simulink model "ARDroneHover_V2_ALTER_D"  (R2026a)
settings: Solver=ode1  StopTime=Inf  FixedStep=sampleTime  EnableMultiTasking=on
values from neighbouring files (symbols this model uses):
  sampleTime = 1/200    (= 0.005)    [Copy_of_setupHover_EXEC_D.m]    (also in Copy_of_setupHover_EXEC_E.m; setupHover.m; setupWPTracking.m)
undefined symbols (not defined in the file or in its folder): Standard_Devices, UDP_Protocol
libraries: sldrtlib x3, dspnetwork x3, aerolibanimutils x1
settings Model: ExtModeTrigDuration=100000  Creator=Paul  LastModifiedBy=vicqu
settings DataIOCC: SignalLoggingSaveFormat=ModelDataLogs  TimeSaveName=time
settings OptimizationCC: InitFltsAndDblsToZero=on
settings DebuggingCC: UnderspecifiedInitializationDetection=Classic
settings HardwareCC: ProdBitPerLong=64.0  ProdHWDeviceType=Intel->x86-64 (Mac OS X)
settings RTWCC: SystemTargetFile=sldrt.tlc  TemplateMakefile=sldrt.tmf  RTWCompilerOptimization=on  Description=Simulink Desktop Real-Time
settings CodeAppCC: MaxIdLength=95.0
settings STFCustomTargetCC: SystemTargetFile=sldrt.tlc  MultiwordLength=2048.0  ModelReferenceCompliant=off  MATLABClassNameForMDSCustomization=Simulink.SoftwareTarget.TargetSpecificTriggerConfigurationBase
settings SimulinkDesktopRealTimeCC: TargetPreCompLibLocation=/Applications/MATLAB_R2017b.app/toolbox/sldrt/lib/maci64  TargetLangStandard=C89/C90 (ANSI)  SupportVariableSizeSignals=off

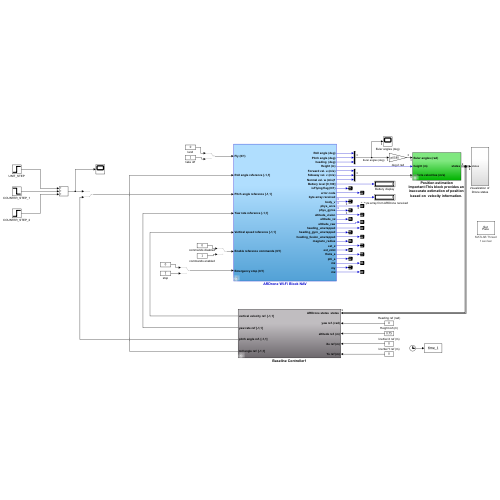
[thumbnail: Simulink's stored preview of the top-level diagram]
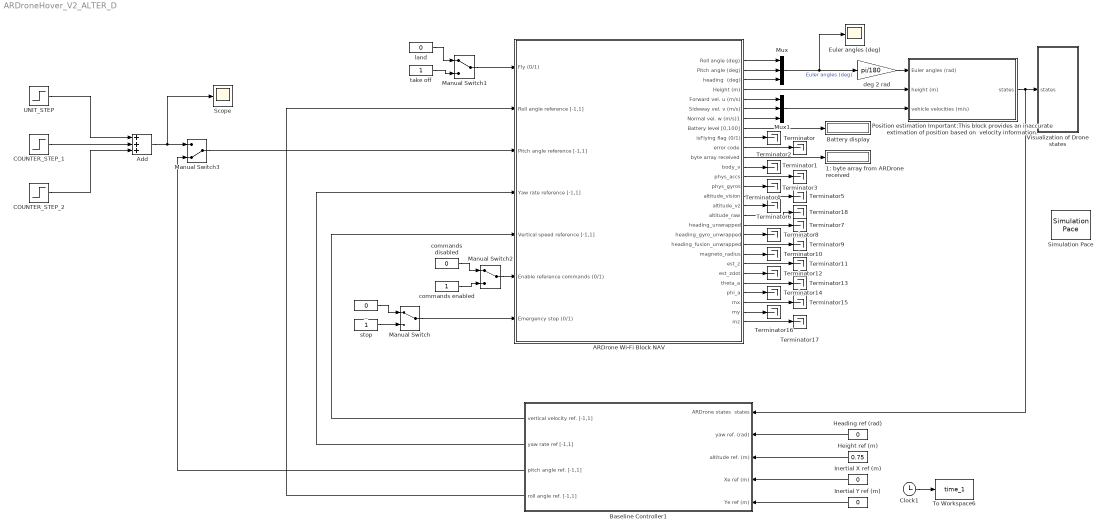
== system ARDroneHover_V2_ALTER_D ==
  "1: byte array from ARDrone received " : Display
  ARDrone Wi-Fi Block NAV : Subsystem  AncestorBlock=ARBlocks/ARDrone Wi-Fi Block NAV
  Add : Sum  Inputs=+++
  Baseline Controller1 : Subsystem  AncestorBlock=ARBlocks/Baseline Controller
  Battery display : Display
  COUNTER_STEP_1 : Step  Time=24  FinalValue=-2  SampleTime=0
  COUNTER_STEP_2 : Step  Time=28  SampleTime=0
  Clock1 : Clock
  Euler angles (deg) : Scope
      settings: ActiveDisplayYMinimum=-141.77037  ActiveDisplayYMaximum=21.99337  DataLoggingMaxPoints=500000
  Heading ref (rad) : Constant  Value=0
  Height ref (m) : Constant  Value=0.75
  Inertial X ref (m) : Constant  Value=0
  Inertial Y ref (m) : Constant  Value=0
  Manual Switch : ManualSwitch
  Manual Switch1 : ManualSwitch
  Manual Switch2 : ManualSwitch
  Manual Switch3 : ManualSwitch  CurrentSetting=0
  Mux : Mux  Inputs=3
  Mux1 : Mux  Inputs=3
  "Position estimation Important:This block provides an inaccurate extimation of position based on  velocity information. " : Subsystem  AncestorBlock=|
      | ARBlocks/Position estimation
      | Important:This block provides an 
      | inaccurate extimation of position 
      | based on  velocity information.
  Scope : Scope
      settings: ActiveDisplayYMinimum=-1  ActiveDisplayYMaximum=1
  Simulation Pace : aerolibanimutils/Simulation Pace  SimulationPace=1  SleepMode=MATLAB Thread  OutputPaceError=off  SampleTime=sampleTime
  Terminator{,1..18} (19 alike) : Terminator
  To Workspace6 : ToWorkspace  VariableName=time_1  SampleTime=sampleTime
  UNIT_STEP : Step  Time=20  SampleTime=0
  Visualization of Drone states : Subsystem
  _ : Constant  Value=0
  commands disabled : Constant  Value=0
  commands enabled : Constant
  deg 2 rad : Gain  Gain=pi/180
  land : Constant  Value=0
  stop : Constant
  take off : Constant
  wires:
  _/1 -> Manual Switch/1
  stop/1 -> Manual Switch/2
  land/1 -> Manual Switch1/1
  take off/1 -> Manual Switch1/2
  commands disabled/1 -> Manual Switch2/1
  commands enabled/1 -> Manual Switch2/2
  Manual Switch1/1 -> ARDrone Wi-Fi Block NAV/1(Fly (0/1))
  Manual Switch2/1 -> ARDrone Wi-Fi Block NAV/6(Enable reference commands (0/1))
  Manual Switch/1 -> ARDrone Wi-Fi Block NAV/7(Emergency stop (0/1))
  ARDrone Wi-Fi Block NAV/1(Roll angle (deg)) -> Mux/1
  ARDrone Wi-Fi Block NAV/2(Pitch angle (deg)) -> Mux/2
  ARDrone Wi-Fi Block NAV/5(Forward vel. u (m/s)) -> Mux1/1
  ARDrone Wi-Fi Block NAV/6(Sideway vel. v (m/s)) -> Mux1/2
  ARDrone Wi-Fi Block NAV/7(Normal vel. w (m/s)1) -> Mux1/3
  Mux/1 -> deg 2 rad/1, Euler angles (deg)/1  "Euler angles (deg)"
  ARDrone Wi-Fi Block NAV/8(Battery level [0,100]) -> Battery display/1
  Baseline Controller1/1(vertical velocity ref. [-1,1]) -> ARDrone Wi-Fi Block NAV/5(Vertical speed reference [-1,1])
  "Position estimation Important:This block provides an inaccurate extimation of position based on  velocity information. "/1(states) -> Baseline Controller1/1("ARDrone states  states "), Visualization of Drone states/1(states)
  deg 2 rad/1 -> "Position estimation Important:This block provides an inaccurate extimation of position based on  velocity information. "/1(Euler angles (rad))
  ARDrone Wi-Fi Block NAV/4(Height (m)) -> "Position estimation Important:This block provides an inaccurate extimation of position based on  velocity information. "/2(height (m))
  Mux1/1 -> "Position estimation Important:This block provides an inaccurate extimation of position based on  velocity information. "/3(vehicle velocities (m/s))
  Baseline Controller1/4(roll angle ref. [-1,1]) -> ARDrone Wi-Fi Block NAV/2(Roll angle reference [-1,1])
  ARDrone Wi-Fi Block NAV/3(heading  (deg)) -> Mux/3
  ARDrone Wi-Fi Block NAV/9(isFlying flag (0/1)) -> Terminator/1
  ARDrone Wi-Fi Block NAV/10(error code) -> Terminator1/1
  ARDrone Wi-Fi Block NAV/11(byte array received) -> "1: byte array from ARDrone received "/1
  Baseline Controller1/2(yaw rate ref [-1,1]) -> ARDrone Wi-Fi Block NAV/4(Yaw rate reference [-1,1])
  Clock1/1 -> To Workspace6/1
  Height ref (m)/1 -> Baseline Controller1/3(altitude ref. (m))
  Inertial X ref (m)/1 -> Baseline Controller1/4(Xe ref (m))
  Inertial Y ref (m)/1 -> Baseline Controller1/5(Ye ref (m))
  Heading ref (rad)/1 -> Baseline Controller1/2(yaw ref. (rad))
  ARDrone Wi-Fi Block NAV/17(altitude_raw) -> Terminator18/1
  ARDrone Wi-Fi Block NAV/12(body_v) -> Terminator2/1
  ARDrone Wi-Fi Block NAV/13(phys_accs) -> Terminator3/1
  ARDrone Wi-Fi Block NAV/14(phys_gyros) -> Terminator4/1
  ARDrone Wi-Fi Block NAV/15(altitude_vision) -> Terminator5/1
  ARDrone Wi-Fi Block NAV/16(altitude_vz) -> Terminator6/1
  ARDrone Wi-Fi Block NAV/19(heading_gyro_unwrapped) -> Terminator8/1
  ARDrone Wi-Fi Block NAV/18(heading_unwrapped) -> Terminator7/1
  ARDrone Wi-Fi Block NAV/21(magneto_radius) -> Terminator10/1
  ARDrone Wi-Fi Block NAV/20(heading_fusion_unwrapped) -> Terminator9/1
  ARDrone Wi-Fi Block NAV/23(est_zdot) -> Terminator12/1
  ARDrone Wi-Fi Block NAV/22(est_z) -> Terminator11/1
  ARDrone Wi-Fi Block NAV/25(phi_a) -> Terminator14/1
  ARDrone Wi-Fi Block NAV/24(theta_a) -> Terminator13/1
  ARDrone Wi-Fi Block NAV/27(my) -> Terminator16/1
  ARDrone Wi-Fi Block NAV/26(mx) -> Terminator15/1
  ARDrone Wi-Fi Block NAV/28(mz) -> Terminator17/1
  Manual Switch3/1 -> ARDrone Wi-Fi Block NAV/3(Pitch angle reference [-1,1])
  Baseline Controller1/3(pitch angle ref. [-1,1]) -> Manual Switch3/2
  Add/1 -> Scope/1, Manual Switch3/1
  UNIT_STEP/1 -> Add/1
  COUNTER_STEP_1/1 -> Add/2
  COUNTER_STEP_2/1 -> Add/3

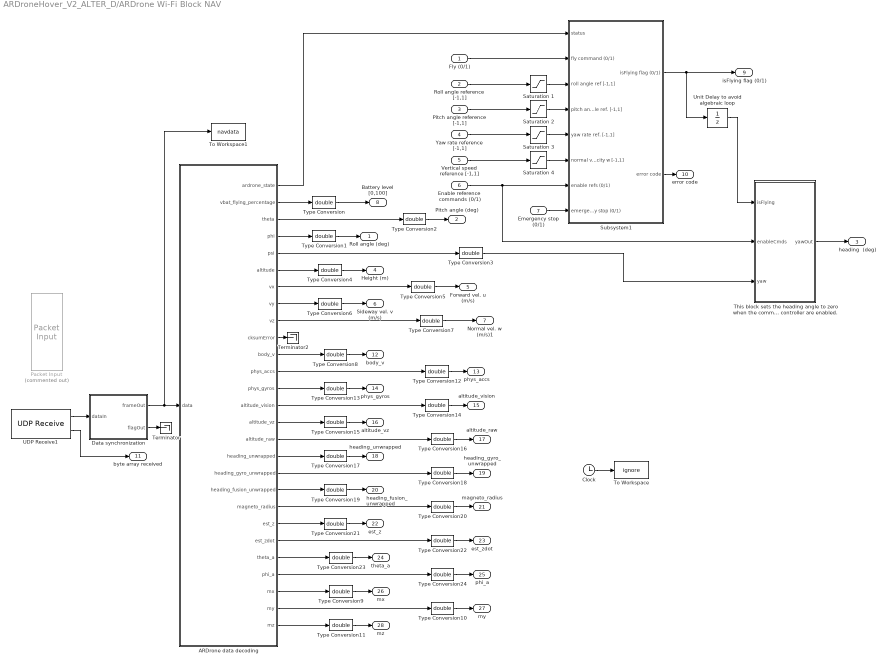
== system ARDroneHover_V2_ALTER_D/ARDrone Wi-Fi Block NAV ==
  Fly (0/1) : Inport
  Roll angle reference [-1,1] : Inport  Port=2
  Pitch angle reference [-1,1] : Inport  Port=3
  Yaw rate reference [-1,1] : Inport  Port=4
  Vertical speed reference [-1,1] : Inport  Port=5
  Enable reference commands (0/1) : Inport  Port=6
  Emergency stop (0/1) : Inport  Port=7
  ARDrone data decoding : MATLAB Function  TreatAsAtomicUnit=on
  Clock : Clock
      settings: Decimation=100
  "Data synchronization " : MATLAB Function  TreatAsAtomicUnit=on
  Packet Input : sldrtlib/Packet Input  Commented=on  SampleTime=sampleTime  MaxMissedTicks=100  ShowMissedTicks=off  YieldWhenWaiting=off  DrvName=Standard_Devices/UDP_Protocol  DrvAddress=5554  DrvOptions=[3232235777 5554]  PacketSize=2190  DataTypes='2190*uint8'  ShowReady=on  ShowError=off  PacketID=1  ByteOrder=1  ShowTimestamp=off
      settings: AttributesFormatString=UDP Protocol [5554]
  Saturation {1..4} (4 alike) : Saturate  UpperLimit=1  LowerLimit=-1
  Subsystem1 : Subsystem
  Terminator : Terminator
  Terminator2 : Terminator
  "This block sets the heading angle to zero when the commands from the Simulink controller are enabled. " : MATLAB Function  TreatAsAtomicUnit=on
  To Workspace : ToWorkspace  VariableName=ignore  SaveFormat=Timeseries  SampleTime=-1
  To Workspace1 : ToWorkspace  VariableName=navdata  SaveFormat=Structure With Time  SampleTime=-1
  Type Conversion{,1..24} (25 alike) : DataTypeConversion  OutDataTypeStr=double  SaturateOnIntegerOverflow=off  RndMeth=Floor
  UDP Receive1 : dspnetwork/UDP Receive  localURL='0.0.0.0'  localPort=5554  remoteURL='192.168.1.1'  remotePort=-1  recvBufferSize=8192  dims=2190  signalDatatype=uint8  isComplex=off  isVarSize=off  showBlockingTime=off  blockingTime=0  sampletime=sampleTime  blockPlatform=[]
  Unit Delay to avoid algebraic loop : UnitDelay  SampleTime=-1
  Roll angle (deg) : Outport  VectorParamsAs1DForOutWhenUnconnected=off
  Pitch angle (deg) : Outport  Port=2  VectorParamsAs1DForOutWhenUnconnected=off
  heading  (deg) : Outport  Port=3  VectorParamsAs1DForOutWhenUnconnected=off
  Height (m) : Outport  Port=4  VectorParamsAs1DForOutWhenUnconnected=off
  Forward vel. u (m/s) : Outport  Port=5  VectorParamsAs1DForOutWhenUnconnected=off
  Sideway vel. v (m/s) : Outport  Port=6  VectorParamsAs1DForOutWhenUnconnected=off
  Normal vel. w (m/s)1 : Outport  Port=7  VectorParamsAs1DForOutWhenUnconnected=off
  Battery level [0,100] : Outport  Port=8  VectorParamsAs1DForOutWhenUnconnected=off
  isFlying flag (0/1) : Outport  Port=9  VectorParamsAs1DForOutWhenUnconnected=off
  error code : Outport  Port=10  VectorParamsAs1DForOutWhenUnconnected=off
  byte array received : Outport  Port=11  VectorParamsAs1DForOutWhenUnconnected=off
  body_v : Outport  Port=12  VectorParamsAs1DForOutWhenUnconnected=off
  phys_accs : Outport  Port=13  VectorParamsAs1DForOutWhenUnconnected=off
  phys_gyros : Outport  Port=14  VectorParamsAs1DForOutWhenUnconnected=off
  altitude_vision : Outport  Port=15  VectorParamsAs1DForOutWhenUnconnected=off
  altitude_vz : Outport  Port=16  VectorParamsAs1DForOutWhenUnconnected=off
  altitude_raw : Outport  Port=17  VectorParamsAs1DForOutWhenUnconnected=off
  heading_unwrapped : Outport  Port=18  VectorParamsAs1DForOutWhenUnconnected=off
  heading_gyro_unwrapped : Outport  Port=19  VectorParamsAs1DForOutWhenUnconnected=off
  heading_fusion_unwrapped : Outport  Port=20  VectorParamsAs1DForOutWhenUnconnected=off
  magneto_radius : Outport  Port=21  VectorParamsAs1DForOutWhenUnconnected=off
  est_z : Outport  Port=22  VectorParamsAs1DForOutWhenUnconnected=off
  est_zdot : Outport  Port=23  VectorParamsAs1DForOutWhenUnconnected=off
  theta_a : Outport  Port=24  VectorParamsAs1DForOutWhenUnconnected=off
  phi_a : Outport  Port=25  VectorParamsAs1DForOutWhenUnconnected=off
  mx : Outport  Port=26  VectorParamsAs1DForOutWhenUnconnected=off
  my : Outport  Port=27  VectorParamsAs1DForOutWhenUnconnected=off
  mz : Outport  Port=28  VectorParamsAs1DForOutWhenUnconnected=off
  wires:
  ARDrone data decoding/27(mz) -> Type Conversion11/1
  Type Conversion11/1 -> mz/1
  ARDrone data decoding/26(my) -> Type Conversion10/1
  Type Conversion10/1 -> my/1
  ARDrone data decoding/25(mx) -> Type Conversion9/1
  Type Conversion9/1 -> mx/1
  ARDrone data decoding/24(phi_a) -> Type Conversion24/1
  ARDrone data decoding/23(theta_a) -> Type Conversion23/1
  ARDrone data decoding/22(est_zdot) -> Type Conversion22/1
  ARDrone data decoding/21(est_z) -> Type Conversion21/1
  ARDrone data decoding/20(magneto_radius) -> Type Conversion20/1
  ARDrone data decoding/19(heading_fusion_unwrapped) -> Type Conversion19/1
  ARDrone data decoding/18(heading_gyro_unwrapped) -> Type Conversion18/1
  ARDrone data decoding/17(heading_unwrapped) -> Type Conversion17/1
  ARDrone data decoding/16(altitude_raw) -> Type Conversion16/1
  ARDrone data decoding/15(altitude_vz) -> Type Conversion15/1
  ARDrone data decoding/14(altitude_vision) -> Type Conversion14/1
  ARDrone data decoding/13(phys_gyros) -> Type Conversion13/1
  ARDrone data decoding/12(phys_accs) -> Type Conversion12/1
  ARDrone data decoding/11(body_v) -> Type Conversion8/1
  ARDrone data decoding/10(cksumError) -> Terminator2/1
  ARDrone data decoding/9(vz) -> Type Conversion7/1
  ARDrone data decoding/8(vy) -> Type Conversion6/1
  ARDrone data decoding/7(vx) -> Type Conversion5/1
  ARDrone data decoding/6(altitude) -> Type Conversion4/1
  ARDrone data decoding/5(psi) -> Type Conversion3/1
  ARDrone data decoding/4(phi) -> Type Conversion1/1
  ARDrone data decoding/3(theta) -> Type Conversion2/1
  ARDrone data decoding/2(vbat_flying_percentage) -> Type Conversion/1
  Type Conversion24/1 -> phi_a/1
  Type Conversion23/1 -> theta_a/1
  Type Conversion22/1 -> est_zdot/1
  Type Conversion21/1 -> est_z/1
  Type Conversion20/1 -> magneto_radius/1
  Type Conversion19/1 -> heading_fusion_unwrapped/1
  Type Conversion18/1 -> heading_gyro_unwrapped/1
  Type Conversion17/1 -> heading_unwrapped/1
  Type Conversion16/1 -> altitude_raw/1
  Type Conversion15/1 -> altitude_vz/1
  Type Conversion14/1 -> altitude_vision/1
  Type Conversion13/1 -> phys_gyros/1
  Type Conversion12/1 -> phys_accs/1
  Type Conversion8/1 -> body_v/1
  Clock/1 -> To Workspace/1
  Unit Delay to avoid algebraic loop/1 -> "This block sets the heading angle to zero when the commands from the Simulink controller are enabled. "/1(isFlying)
  "Data synchronization "/2(flagOut) -> Terminator/1
  Saturation 4/1 -> Subsystem1/6(normal velocity w [-1,1])
  Saturation 3/1 -> Subsystem1/5(yaw rate ref. [-1,1])
  Saturation 2/1 -> Subsystem1/4(pitch angle ref. [-1,1])
  Saturation 1/1 -> Subsystem1/3(roll angle ref [-1,1])
  Fly (0/1)/1 -> Subsystem1/2(fly command (0/1))
  "This block sets the heading angle to zero when the commands from the Simulink controller are enabled. "/1(yawOut) -> heading  (deg)/1
  Type Conversion3/1 -> "This block sets the heading angle to zero when the commands from the Simulink controller are enabled. "/3(yaw)
  Type Conversion7/1 -> Normal vel. w (m/s)1/1
  Type Conversion6/1 -> Sideway vel. v (m/s)/1
  Type Conversion5/1 -> Forward vel. u (m/s)/1
  Type Conversion4/1 -> Height (m)/1
  Type Conversion2/1 -> Pitch angle (deg)/1
  Type Conversion1/1 -> Roll angle (deg)/1
  Type Conversion/1 -> Battery level [0,100]/1
  Subsystem1/2(error code) -> error code/1
  Subsystem1/1(isFlying flag (0/1)) -> Unit Delay to avoid algebraic loop/1, isFlying flag (0/1)/1
  Emergency stop (0/1)/1 -> Subsystem1/8(emergency stop (0/1))
  Enable reference commands (0/1)/1 -> Subsystem1/7(enable refs (0/1)), "This block sets the heading angle to zero when the commands from the Simulink controller are enabled. "/2(enableCmds)
  Vertical speed reference [-1,1]/1 -> Saturation 4/1
  Yaw rate reference [-1,1]/1 -> Saturation 3/1
  Pitch angle reference [-1,1]/1 -> Saturation 2/1
  Roll angle reference [-1,1]/1 -> Saturation 1/1
  ARDrone data decoding/1(ardrone_state) -> Subsystem1/1(status)
  UDP Receive1/2 -> byte array received/1
  "Data synchronization "/1(frameOut) -> To Workspace1/1, ARDrone data decoding/1(data)
  UDP Receive1/1 -> "Data synchronization "/1(dataIn)

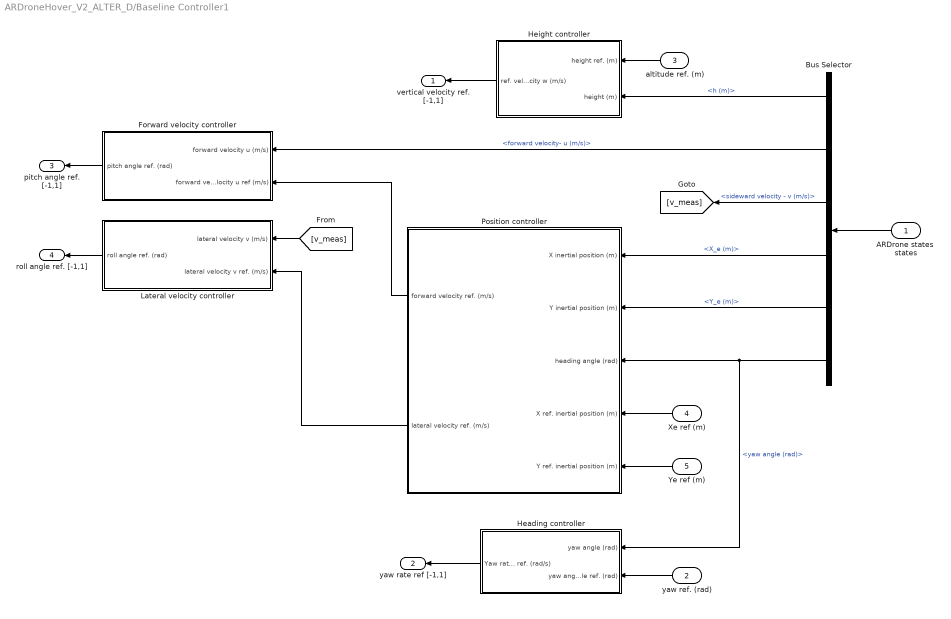
== system ARDroneHover_V2_ALTER_D/Baseline Controller1 ==
  "ARDrone states  states " : Inport
  yaw ref. (rad) : Inport  Port=2
  altitude ref. (m) : Inport  Port=3
  Xe ref (m) : Inport  Port=4
  Ye ref (m) : Inport  Port=5
  Bus Selector : BusSelector  OutputSignals=h (m),forward velocity- u (m/s),sideward velocity - v (m/s),X_e (m),Y_e (m),yaw angle (rad)
  "Forward velocity controller " : Subsystem
  Heading controller : Subsystem
  "Height controller " : Subsystem
  Lateral velocity controller : Subsystem
  Position controller : Subsystem
  vertical velocity ref. [-1,1] : Outport  VectorParamsAs1DForOutWhenUnconnected=off
  yaw rate ref [-1,1] : Outport  Port=2  VectorParamsAs1DForOutWhenUnconnected=off
  pitch angle ref. [-1,1] : Outport  Port=3  VectorParamsAs1DForOutWhenUnconnected=off
  roll angle ref. [-1,1] : Outport  Port=4  VectorParamsAs1DForOutWhenUnconnected=off
  wires:
  [v_meas] -> Lateral velocity controller/1(lateral velocity v (m/s))
  Bus Selector/3 -> [v_meas]  "<sideward velocity - v (m/s)>"
  Position controller/2(lateral velocity ref. (m/s)) -> Lateral velocity controller/2(lateral velocity v ref. (m/s))
  Position controller/1(forward velocity ref. (m/s)) -> "Forward velocity controller "/2(forward velocity u ref (m/s))
  Ye ref (m)/1 -> Position controller/5(Y ref. inertial position (m))
  Xe ref (m)/1 -> Position controller/4(X ref. inertial position (m))
  Bus Selector/5 -> Position controller/2(Y inertial position (m))  "<Y_e (m)>"
  Bus Selector/4 -> Position controller/1(X inertial position (m))  "<X_e (m)>"
  Heading controller/1(Yaw rate ref. (rad/s)) -> yaw rate ref [-1,1]/1
  yaw ref. (rad)/1 -> Heading controller/2(yaw angle ref. (rad))
  "Forward velocity controller "/1(pitch angle ref. (rad)) -> pitch angle ref. [-1,1]/1
  Bus Selector/2 -> "Forward velocity controller "/1(forward velocity u (m/s))  "<forward velocity- u (m/s)>"
  Lateral velocity controller/1(roll angle ref. (rad)) -> roll angle ref. [-1,1]/1
  "Height controller "/1(ref. velocity w (m/s)) -> vertical velocity ref. [-1,1]/1
  Bus Selector/1 -> "Height controller "/2(height (m))  "<h (m)>"
  altitude ref. (m)/1 -> "Height controller "/1(height ref. (m))
  "ARDrone states  states "/1 -> Bus Selector/1
  Bus Selector/6 -> Position controller/3(heading angle (rad)), Heading controller/1(yaw angle (rad))  "<yaw angle (rad)>"

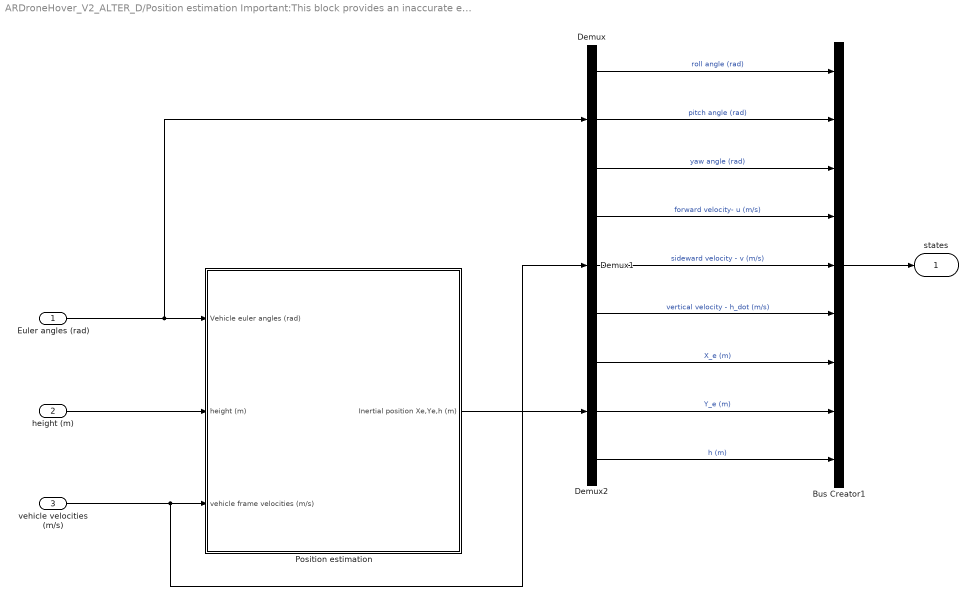
== system ARDroneHover_V2_ALTER_D/Position estimation Important:This block provides an inaccurate extimation of position based on  velocity information.  ==
  Euler angles (rad) : Inport
  height (m) : Inport  Port=2
  vehicle velocities (m/s) : Inport  Port=3
  Bus Creator1 : BusCreator  Inputs=9
  Demux : Demux  Outputs=3
  Demux1 : Demux  Outputs=3
  Demux2 : Demux  Outputs=3
  Position estimation : Subsystem
  states : Outport  VectorParamsAs1DForOutWhenUnconnected=off
  wires:
  height (m)/1 -> Position estimation/2(height (m))
  Bus Creator1/1 -> states/1
  Demux2/3 -> Bus Creator1/9  "h (m)"
  Demux2/2 -> Bus Creator1/8  "Y_e (m)"
  Demux2/1 -> Bus Creator1/7  "X_e (m)"
  Demux1/3 -> Bus Creator1/6  "vertical velocity - h_dot (m/s)"
  Demux1/2 -> Bus Creator1/5  "sideward velocity - v (m/s)"
  Demux1/1 -> Bus Creator1/4  "forward velocity- u (m/s)"
  Demux/3 -> Bus Creator1/3  "yaw angle (rad)"
  Demux/2 -> Bus Creator1/2  "pitch angle (rad)"
  Demux/1 -> Bus Creator1/1  "roll angle (rad)"
  Position estimation/1(Inertial position Xe,Ye,h (m)) -> Demux2/1
  Euler angles (rad)/1 -> Demux/1, Position estimation/1(Vehicle euler angles (rad))
  vehicle velocities (m/s)/1 -> Position estimation/3(vehicle frame velocities (m/s)), Demux1/1

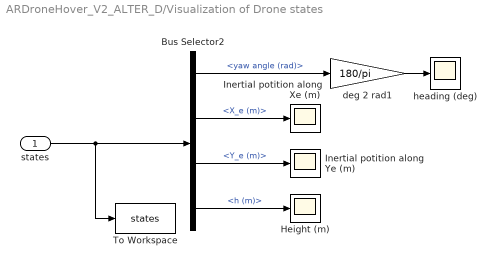
== system ARDroneHover_V2_ALTER_D/Visualization of Drone states ==
  states : Inport
  Bus Selector2 : BusSelector  OutputSignals=yaw angle (rad),X_e (m),Y_e (m),h (m)
  Height (m) : Scope
      settings: ActiveDisplayYMinimum=-1  ActiveDisplayYMaximum=1  DataLoggingMaxPoints=500000  DataLoggingVariableName=ScopeData5
  Inertial potition along Xe (m) : Scope
      settings: ActiveDisplayYMinimum=-22.5  ActiveDisplayYMaximum=22.5  DataLoggingMaxPoints=500000  DataLoggingVariableName=ScopeData3
  Inertial potition along Ye (m) : Scope
      settings: ActiveDisplayYMinimum=-22.5  ActiveDisplayYMaximum=22.5  DataLoggingMaxPoints=500000  DataLoggingVariableName=ScopeData4
  To Workspace : ToWorkspace  VariableName=states  SaveFormat=Structure With Time  SampleTime=-1
  deg 2 rad1 : Gain  Gain=180/pi
  heading (deg) : Scope
      settings: ActiveDisplayYMinimum=-22.5  ActiveDisplayYMaximum=22.5  DataLoggingMaxPoints=500000  DataLoggingVariableName=ScopeData2
  wires:
  states/1 -> To Workspace/1, Bus Selector2/1
  Bus Selector2/1 -> deg 2 rad1/1  "<yaw angle (rad)>"
  Bus Selector2/2 -> Inertial potition along Xe (m)/1  "<X_e (m)>"
  Bus Selector2/3 -> Inertial potition along Ye (m)/1  "<Y_e (m)>"
  Bus Selector2/4 -> Height (m)/1  "<h (m)>"
  deg 2 rad1/1 -> heading (deg)/1

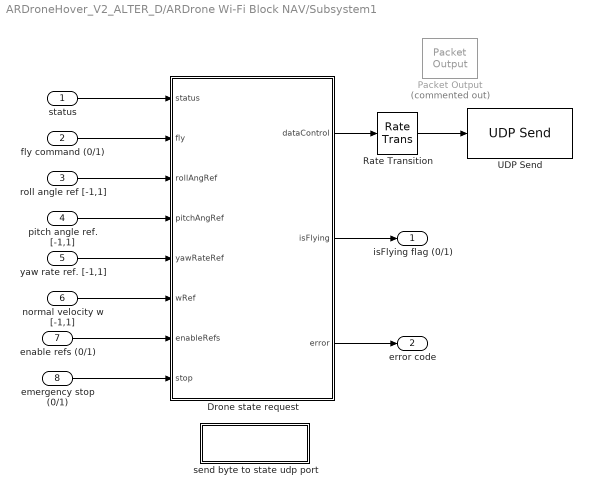
== system ARDroneHover_V2_ALTER_D/ARDrone Wi-Fi Block NAV/Subsystem1 ==
  status : Inport
  fly command (0/1) : Inport  Port=2
  roll angle ref [-1,1] : Inport  Port=3
  pitch angle ref. [-1,1] : Inport  Port=4
  yaw rate ref. [-1,1] : Inport  Port=5
  normal velocity w [-1,1] : Inport  Port=6
  enable refs (0/1) : Inport  Port=7
  emergency stop (0/1) : Inport  Port=8
  Drone state request : MATLAB Function  TreatAsAtomicUnit=on  SystemSampleTime=sampleTime
  Packet Output : sldrtlib/Packet Output  Commented=on  SampleTime=-1  MaxMissedTicks=100  ShowMissedTicks=off  YieldWhenWaiting=off  DrvName=Standard_Devices/UDP_Protocol  DrvAddress=5556  DrvOptions=[3232235777 5556]  PacketSize=150  DataTypes='150*uint8'  ShowReady=off  ShowError=off  PacketID=1  ByteOrder=1  InitialValue=[]  FinalValue=[]
      settings: AttributesFormatString=UDP Protocol [5556]
  Rate Transition : RateTransition  OutPortSampleTime=sampleTime*6
  UDP Send : dspnetwork/UDP Send  remoteURL='192.168.1.1'  remotePort=5556  localURL='0.0.0.0'  localPortSource=Specify via dialog  localPort=5556  sendBufferSize=8192  sampletime=-1  blockPlatform=[]  separateLengthPort=0
  "send byte to state udp port " : Subsystem
  isFlying flag (0/1) : Outport  VectorParamsAs1DForOutWhenUnconnected=off
  error code : Outport  Port=2  VectorParamsAs1DForOutWhenUnconnected=off
  wires:
  Drone state request/3(error) -> error code/1
  emergency stop (0/1)/1 -> Drone state request/8(stop)
  enable refs (0/1)/1 -> Drone state request/7(enableRefs)
  normal velocity w [-1,1]/1 -> Drone state request/6(wRef)
  yaw rate ref. [-1,1]/1 -> Drone state request/5(yawRateRef)
  roll angle ref [-1,1]/1 -> Drone state request/3(rollAngRef)
  Drone state request/2(isFlying) -> isFlying flag (0/1)/1
  Drone state request/1(dataControl) -> Rate Transition/1
  status/1 -> Drone state request/1(status)
  pitch angle ref. [-1,1]/1 -> Drone state request/4(pitchAngRef)
  fly command (0/1)/1 -> Drone state request/2(fly)
  Rate Transition/1 -> UDP Send/1

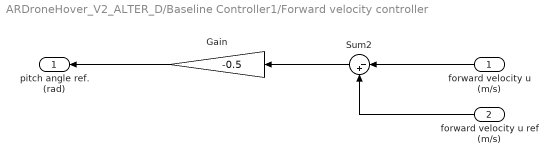
== system ARDroneHover_V2_ALTER_D/Baseline Controller1/Forward velocity controller  ==
  forward velocity u (m/s) : Inport
  forward velocity u ref (m/s) : Inport  Port=2
  Gain : Gain  Gain=-0.5
  Sum2 : Sum  Inputs=|-+
  pitch angle ref. (rad) : Outport  VectorParamsAs1DForOutWhenUnconnected=off
  wires:
  forward velocity u ref (m/s)/1 -> Sum2/2
  Gain/1 -> pitch angle ref. (rad)/1
  Sum2/1 -> Gain/1
  forward velocity u (m/s)/1 -> Sum2/1

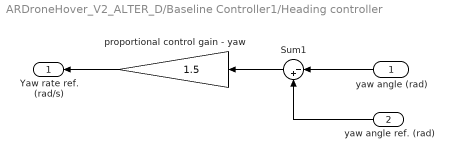
== system ARDroneHover_V2_ALTER_D/Baseline Controller1/Heading controller ==
  yaw angle (rad) : Inport
  yaw angle ref. (rad) : Inport  Port=2
  Sum1 : Sum  Inputs=|-+
  proportional control gain - yaw : Gain  Gain=1.5
  Yaw rate ref. (rad/s) : Outport  VectorParamsAs1DForOutWhenUnconnected=off
  wires:
  yaw angle ref. (rad)/1 -> Sum1/2
  Sum1/1 -> proportional control gain - yaw/1
  proportional control gain - yaw/1 -> Yaw rate ref. (rad/s)/1
  yaw angle (rad)/1 -> Sum1/1

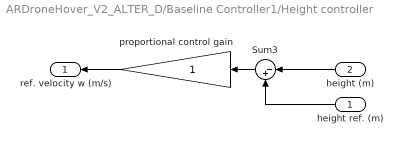
== system ARDroneHover_V2_ALTER_D/Baseline Controller1/Height controller  ==
  height ref. (m) : Inport
  height (m) : Inport  Port=2
  Sum3 : Sum  Inputs=|-+
  proportional control gain : Gain
  ref. velocity w (m/s) : Outport  VectorParamsAs1DForOutWhenUnconnected=off
  wires:
  height ref. (m)/1 -> Sum3/2
  height (m)/1 -> Sum3/1
  Sum3/1 -> proportional control gain/1
  proportional control gain/1 -> ref. velocity w (m/s)/1

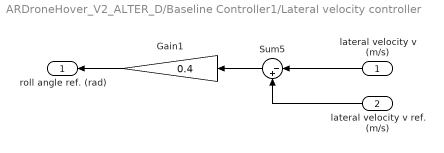
== system ARDroneHover_V2_ALTER_D/Baseline Controller1/Lateral velocity controller ==
  lateral velocity v (m/s) : Inport
  lateral velocity v ref. (m/s) : Inport  Port=2
  Gain1 : Gain  Gain=0.4
  Sum5 : Sum  Inputs=|-+
  roll angle ref. (rad) : Outport  VectorParamsAs1DForOutWhenUnconnected=off
  wires:
  lateral velocity v ref. (m/s)/1 -> Sum5/2
  Gain1/1 -> roll angle ref. (rad)/1
  Sum5/1 -> Gain1/1
  lateral velocity v (m/s)/1 -> Sum5/1

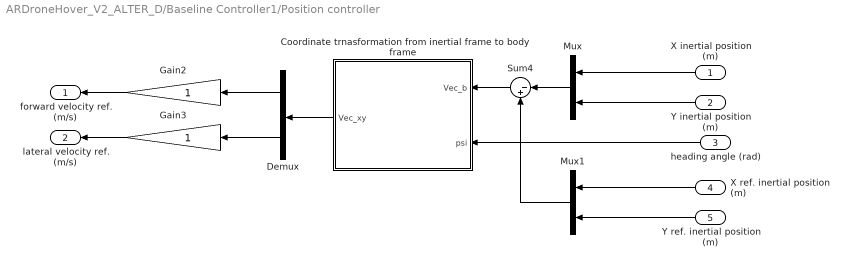
== system ARDroneHover_V2_ALTER_D/Baseline Controller1/Position controller ==
  X inertial position (m) : Inport
  Y inertial position (m) : Inport  Port=2
  heading angle (rad) : Inport  Port=3
  X ref. inertial position (m) : Inport  Port=4
  Y ref. inertial position (m) : Inport  Port=5
  "Coordinate trnasformation from inertial frame to body frame " : MATLAB Function  TreatAsAtomicUnit=on
  Demux : Demux  Outputs=2
  Gain2 : Gain
  Gain3 : Gain
  Mux : Mux  Inputs=2
  Mux1 : Mux  Inputs=2
  Sum4 : Sum  Inputs=|-+
  forward velocity ref. (m/s) : Outport  VectorParamsAs1DForOutWhenUnconnected=off
  lateral velocity ref. (m/s) : Outport  Port=2  VectorParamsAs1DForOutWhenUnconnected=off
  wires:
  Gain3/1 -> lateral velocity ref. (m/s)/1
  Demux/2 -> Gain3/1
  Demux/1 -> Gain2/1
  Y ref. inertial position (m)/1 -> Mux1/2
  X ref. inertial position (m)/1 -> Mux1/1
  Mux/1 -> Sum4/1
  X inertial position (m)/1 -> Mux/1
  Y inertial position (m)/1 -> Mux/2
  Sum4/1 -> "Coordinate trnasformation from inertial frame to body frame "/1(Vec_b)
  Mux1/1 -> Sum4/2
  "Coordinate trnasformation from inertial frame to body frame "/1(Vec_xy) -> Demux/1
  heading angle (rad)/1 -> "Coordinate trnasformation from inertial frame to body frame "/2(psi)
  Gain2/1 -> forward velocity ref. (m/s)/1

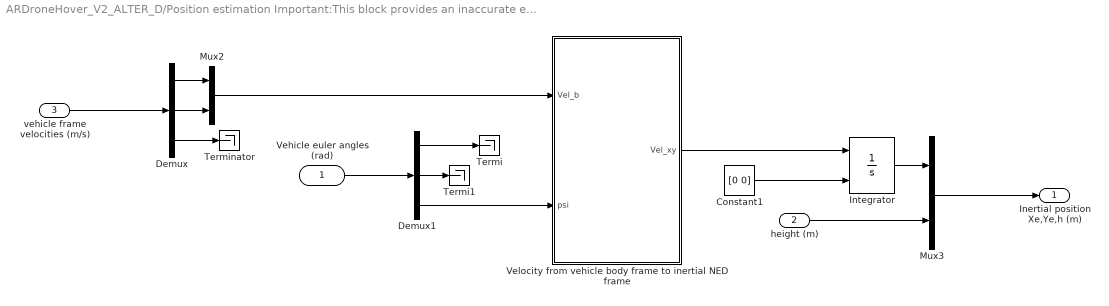
== system ARDroneHover_V2_ALTER_D/Position estimation Important:This block provides an inaccurate extimation of position based on  velocity information. /Position estimation ==
  Vehicle euler angles (rad) : Inport
  height (m) : Inport  Port=2
  vehicle frame velocities (m/s) : Inport  Port=3
  Constant1 : Constant  Value=[0 0]
  Demux : Demux  Outputs=3
  Demux1 : Demux  Outputs=3
  Integrator : Integrator  InitialConditionSource=external
  Mux2 : Mux  Inputs=2
  Mux3 : Mux  Inputs=2
  Termi : Terminator
  Termi1 : Terminator
  Terminator : Terminator
  Velocity from vehicle body frame to inertial NED  frame : MATLAB Function  TreatAsAtomicUnit=on
  Inertial position Xe,Ye,h (m) : Outport  VectorParamsAs1DForOutWhenUnconnected=off
  wires:
  Mux3/1 -> Inertial position Xe,Ye,h (m)/1
  height (m)/1 -> Mux3/2
  Vehicle euler angles (rad)/1 -> Demux1/1
  vehicle frame velocities (m/s)/1 -> Demux/1
  Demux1/3 -> Velocity from vehicle body frame to inertial NED  frame/2(psi)
  Integrator/1 -> Mux3/1
  Constant1/1 -> Integrator/2
  Velocity from vehicle body frame to inertial NED  frame/1(Vel_xy) -> Integrator/1
  Demux1/2 -> Termi1/1
  Demux1/1 -> Termi/1
  Mux2/1 -> Velocity from vehicle body frame to inertial NED  frame/1(Vel_b)
  Demux/1 -> Mux2/1
  Demux/2 -> Mux2/2
  Demux/3 -> Terminator/1

== system ARDroneHover_V2_ALTER_D/ARDrone Wi-Fi Block NAV/Subsystem1/send byte to state udp port  ==
  Constant : Constant  Value=[1 ;13]  OutDataTypeStr=uint8
  Packet Output1 : sldrtlib/Packet Output  Commented=on  SampleTime=sampleTime*10  MaxMissedTicks=100  ShowMissedTicks=off  YieldWhenWaiting=off  DrvName=Standard_Devices/UDP_Protocol  DrvAddress=5554  DrvOptions=[3232235777 5554]  PacketSize=2  DataTypes='2*uint8'  ShowReady=off  ShowError=off  PacketID=1  ByteOrder=1  InitialValue=[]  FinalValue=[]
      settings: AttributesFormatString=UDP Protocol [5554]
  Rate Transition : RateTransition  OutPortSampleTime=sampleTime*10
  UDP Send : dspnetwork/UDP Send  remoteURL='192.168.1.1'  remotePort=5554  localURL='0.0.0.0'  localPortSource=Specify via dialog  localPort=5554  sendBufferSize=8192  sampletime=-1  blockPlatform=[]  separateLengthPort=0
  wires:
  Rate Transition/1 -> UDP Send/1
  Constant/1 -> Rate Transition/1

== matlab function ARDroneHover_V2_ALTER_D/ARDrone Wi-Fi Block NAV/Data synchronization  ==
  data: dataIn input; frameOut output; flagOut output
function [frameOut,flagOut]  = fcn(dataIn)
%#eml
%% Author: David Escobar Sanabria
%  Description: This function synchronizes data coming from the flight computer
%  computer. 
%  frameOut: Organized frame
%  frameIn: sequence of bytes not sync.
persistent frame; 
persistent lastFrame; 
persistent count; 
persistent countHeader; 
persistent countBuffer; 
persistent buffer; 

%% Size of byte array containing the data
sizePayload= 2186;

%% Size of the array read each time step
nBytes = 2190 ;%size(dataIn,1); 


%%%%%%%%%%%%%%%%%%%%%%%%%%%%%%%%%%%%%%%%%%%%%%%%%%%%%%%
%% Initialization of presistent variables
if isempty(buffer)
    buffer=uint8(zeros(10000,1));
end

if isempty(countBuffer)
    countBuffer=0;
end


if isempty(frame)
    frame=uint8(zeros(sizePayload,1));
end

if isempty(lastFrame)
    lastFrame=uint8(zeros(sizePayload,1));
end


if isempty(count)
    count=0;
end

if isempty(countHeader)
    countHeader=0;
end
%%%%%%%%%%%%%%%%%%%%%%%%%%%%%%%%%%%%%%%%%%%%%%%%%%%%%%%

%% Filling the buffer
buffer(countBuffer+1:countBuffer+nBytes) = dataIn;

bytesToRead = countBuffer+nBytes; 

%%%%%%%%%%%%%%%%%%%%%%%%%%%%%%%%%%%%%%%%%%%%%%%%%%%%%%%
%% Reading buffer

for k=1:bytesToRead    
    if(countHeader==4 && count<sizePayload)
        bytesLeft = sizePayload-count;
        frame(count+1:sizePayload) = buffer(k:k+bytesLeft-1);
        count = sizePayload;
        countBuffer = bytesToRead-bytesLeft ;
        buffer(1:countBuffer) = buffer(k+bytesLeft:bytesToRead);
        break;
        
    end
    
    if(countHeader==3 && buffer(k)==85)
        
        countHeader=4;
 
        if(bytesToRead-k > sizePayload)
            count =sizePayload;  
            frame(1:count) = buffer(k+1:k+sizePayload);  
            countBuffer =bytesToRead-k-sizePayload ; 
            buffer(1:countBuffer) = buffer(k+sizePayload+1:bytesToRead);
        else
            
            count =bytesToRead-k;
            if count > 0          
                frame(1:count) = buffer(k+1:bytesToRead);  
            end
            countBuffer = 0; 
            
        end
        
        break;
    end
    
    if(countHeader==2 && buffer(k)==102)
        countHeader=3;
    end
    
    if(countHeader==1 && buffer(k)==119)
        countHeader=2;
    end
       
    if(countHeader==0 && buffer(k)==136)
        countHeader=1;
    end

end

if count==sizePayload 
     frameOut = frame(1:sizePayload,1); % forcei tamanho maximo...
     flagOut = 1; 
     lastFrame = frame;
     frame=uint8(zeros(sizePayload,1));
     count=0;
     countHeader=0;
     
else % In case the buffer does not have an entire payload
    frameOut = lastFrame;
    flagOut = 0; 
end

== matlab function ARDroneHover_V2_ALTER_D/ARDrone Wi-Fi Block NAV/Subsystem1/Drone state request ==
  data: status input; fly input; rollAngRef input; pitchAngRef input; yawRateRef input; wRef input; enableRefs input; dataControl output; isFlying output; stop input; error output
function [dataControl, isFlying, error] = fcn( status, fly, rollAngRef, pitchAngRef, yawRateRef, wRef, enableRefs, stop)
%#codegen

% Persistent variables.
persistent SequenceNumber ;

% Initialization of persistent variables at first time step. 

if isempty(SequenceNumber)
    SequenceNumber = 1 ;
end



% Error code / No error: 0
error=0;

% Boolean of flying status / Flying: 1
isFlying = status(32) ;

% Byte array of size 150 to be sent to the drone.
strOut = uint8(zeros(150,1)) ;

% String that coontains a variable size command. 
% cmd is concatenated with previous commands at each sample
cmd = '';

% At first time step and every 100 time steps, data is requested.
if (SequenceNumber <=1 || mod(SequenceNumber, 100) ==0 )
    SequenceNumber = SequenceNumber+1; 
    strCmd = getString(SequenceNumber) ;
    cmd = ['AT*CONFIG=' strCmd ',"general:navdata_demo","FALSE"' char(13)];
    
end

SequenceNumber = SequenceNumber+1;
strCmd = getString(SequenceNumber) ;
cmd = [cmd 'AT*COMWDG=' strCmd char(13)];


if stop ==1 % Emergency stop
   cmd = ['AT*REF=' strCmd ',290717952' char(13)] ; 
    
else % Not emergency stop
    
    if SequenceNumber >20 && SequenceNumber <22
        
        % Trim vehicle state estimation / angles set to zero
        SequenceNumber =SequenceNumber+1;
        strCmd = getString(SequenceNumber) ;
        cmd = [cmd 'AT*FTRIM=' strCmd char(13)] ;
        
    elseif SequenceNumber >=22 && SequenceNumber <25
        cmd = [cmd 'AT*CONFIG=' strCmd '"conrol:altitude_max","100000"' char(13)] ;
        
        
    elseif SequenceNumber >=25
        
        if ( fly == 1  )
            
            if (isFlying ==0)
                
                SequenceNumber =SequenceNumber+1;
                strCmd = getString(SequenceNumber) ;
                cmd = [cmd 'AT*REF=' strCmd ',290718208' char(13)] ;
                
            elseif isFlying==1 && enableRefs==1
                
                SequenceNumber =SequenceNumber+1;
                strCmd = getString(SequenceNumber) ;
                      
                cmd = [cmd 'AT*PCMD=' strCmd ',1,'] ;
                 
                aux = double (float2IEEE754 (rollAngRef) )  ;
                strAux = getString(abs(aux)) ; 
                if rollAngRef<0
                   strAux = [char(45) strAux] ; 
                end
                cmd = [cmd strAux ','];
                      
               aux = double (float2IEEE754 (pitchAngRef) ) ;
               strAux = getString(abs(aux)) ; 
               if pitchAngRef<0
                    strAux = [char(45) strAux] ; 
               end
               cmd = [cmd strAux ','];
                      
               aux =  double(float2IEEE754 (wRef)) ;
               strAux = getString(abs(aux)) ; 
               if wRef<0
                    strAux = [char(45) strAux] ; 
               end
               cmd = [cmd strAux ','];
                      
                      
               aux =  double (float2IEEE754 (yawRateRef) ) ;
               strAux = getString(abs(aux)) ; 
               if yawRateRef <0
                     error=2; 
                     strAux = [char(45) strAux] ; 
               end
               cmd = [cmd strAux char(13)];
               
                
            end
            
            
        elseif ( fly==0 )
                
               if isFlying ==1
                    SequenceNumber =SequenceNumber+1;
                    strCmd = getString(SequenceNumber) ;
                    cmd = [cmd 'AT*REF=' strCmd ',290717696' char(13)] ;
                    
               end
        end
        
    end
    
%     SequenceNumber =SequenceNumber+1;
%     strCmd = getString(SequenceNumber) ;
%     cmd = [cmd 'AT*PWM=' strCmd ',0,0,0,0'] ;
    
end

% cmd must contain less than 150 bytes. 
if (length(cmd)<150)
    strOut(1:length(cmd)) = cmd ;
else
    error =1; 
end

dataControl = strOut;

end


%% My str2num function that allows for code generation
function [ strOut] = getString( a )
d=1;

if (a<10)
    d=1;
end

if (a >=10 && a <100)
    d=2;
end

if (a >=100 && a <1000)
    d=3;
end

if (a >=1000 && a <10000)
    d=4;
end

if (a >=10000 && a <100000)
    d=5;
end

if (a >=100000 && a <1000000)
    d=6;
end

if (a >=1000000 && a <10000000)
    d=7;
end

if (a >=10000000 && a <100000000)
    d=8;
end

if (a >=100000000 && a <1000000000)
    d=9;
end

if (a >=1000000000 && a <10000000000)
    d=10;
end

if (a >=10000000000 )
    d=11;
end



digit = uint8(zeros(1,d)) ;
resTotal = 0;
%d = length(a) ;
for k=1:d
    
    res1 = mod(a,10^k)/(10^(k-1)) ;
    %( mod(a,10*k) - resTotal)/(10*k) ;
    
    digit(d-k+1) = char(48 + res1);
    resTotal = (10^(k-1))*res1 +resTotal;
    
end

strOut = char(digit) ;


end

%% Function to obtain a IEEE754 representation of a float number
function [ iVal ] = float2IEEE754( fVal )

binData = dec2bin(typecast (single(fVal), 'uint8'),8) ;

binData2 =[ binData(4,:) binData(3,:) binData(2,:) binData(1,:)] ;
iVal =0; 
for k=32:-1:1
    
    if (binData2(k) =='1')
        bit = 1;
    else
        bit =0;
    end
    
    if k == 1
        iVal = iVal - bit*2^(31);
    else
        iVal = iVal + bit*2^(32-k) ; 
    end
    
end

iVal = int32(iVal);

end

== matlab function ARDroneHover_V2_ALTER_D/ARDrone Wi-Fi Block NAV/This block sets the heading angle to zero when the commands from the Simulink controller are enabled.  ==
  data: isFlying input; enableCmds input; yawOut output; yaw input
% Description: This function zeroes out the heading angle once the commands
% are enabled. 
function yawOut = fcn(isFlying,enableCmds,yaw)
%#codegen

yawOut = yaw; 
persistent yaw0 ; 
persistent mode ; 

if isempty (yaw0)
yaw0 = 0; 
end


if isempty (mode)
mode=0; 
end

if isFlying ==1 && enableCmds==1    
    yawOut = yaw - yaw0; 
    mode =1; 
elseif isFlying ==1 && mode ==0
    yaw0 = yaw; 
end


yawOut = mod(yawOut, 360) ;
if yawOut > 180
    yawOut = -360 + yawOut ; 
end

== matlab function ARDroneHover_V2_ALTER_D/Position estimation Important:This block provides an inaccurate extimation of position based on  velocity information. /Position estimation/Velocity from vehicle body frame to inertial NED  frame ==
  data: Vel_b input; Vel_xy output; psi input
function Vel_xy = fcn(Vel_b , psi)
%#codegen
T = [cos(psi) -sin(psi) ; sin(psi) cos(psi)] ; 
Vel_xy = T*Vel_b;

== matlab function ARDroneHover_V2_ALTER_D/Baseline Controller1/Position controller/Coordinate trnasformation from inertial frame to body frame  ==
  data: Vec_b input; Vec_xy output; psi input
function Vec_xy  = fcn(Vec_b , psi)
%#codegen
T = [cos(psi) sin(psi) ; -sin(psi) cos(psi)] ; 
Vec_xy = T*Vec_b(1:2,1);

== matlab function ARDroneHover_V2_ALTER_D/ARDrone Wi-Fi Block NAV/ARDrone data decoding ==
  data: ardrone_state output; vbat_flying_percentage output; theta output; phi output; psi output; altitude output; vx output; vy output; vz output; cksumError output; body_v output; phys_accs output; phys_gyros output; altitude_vision output; altitude_vz output; altitude_raw output; heading_unwrapped output; heading_gyro_unwrapped output; heading_fusion_unwrapped output; magneto_radius output; est_z output; est_zdot output; theta_a output; phi_a output; mx output; my output; data input; mz output
function [ardrone_state, vbat_flying_percentage,...
    theta, phi, psi, altitude, vx, vy, vz , cksumError, body_v,...
    phys_accs,phys_gyros,altitude_vision,altitude_vz,altitude_raw,heading_unwrapped,heading_gyro_unwrapped,...
    heading_fusion_unwrapped,magneto_radius,est_z,est_zdot,theta_a,phi_a,mx, my, mz]= trata_dados_large(data)

%initialie arrays
phys_accs=zeros(3,1);
phys_gyros=zeros(3,1);
body_v=zeros(3,1);

% Checksum array. cksum(1) contains the computed checksum, cksum(2)
% contains the checksum sent by the ARDrone. 
cksum = [0 0 ]; 

% Computing checksum
cksum(1) =  sum(double(data(1:end-8)))+442; 
% Checksum given by the drone
cksum(2) = double(data(end-3)) + double(data(end-2))*256 +  double(data(end-1))*256^2 + double(data(end))*256^3 ; 
% Checksum error
cksumError = abs(cksum(1)-cksum(2));

% Converting bytes to drone information

% header data
ardrone_state = getDroneState(data(1:4));

% demo data
vbat_flying_percentage = decode_32bit(data(21:24),1); % unit: percentage 0 -100
theta = decode_32bit(data(25:28),0)/1000; % unit: deg
phi = decode_32bit(data(29:32),0)/1000; % unit: deg
psi = decode_32bit(data(33:36),0)/1000; % unit: deg
altitude = double(decode_32bit(data(37:40),1))/1000; % unit: m
vx = decode_32bit(data(41:44),0)/1000; % unit: m/s
vy = decode_32bit(data(45:48),0)/1000; % unit: m/s
vz = decode_32bit(data(49:52),0)/1000; % unit: m/s
detection_camera_type = decode_32bit(data(109:112),1);

phys_accs(1) = decode_32bit(data(231:234),0);
phys_accs(2) = decode_32bit(data(235:238),0);
phys_accs(3) = decode_32bit(data(239:242),0);
phys_gyros(1) = decode_32bit(data(243:246),0);
phys_gyros(2) = decode_32bit(data(247:250),0);
phys_gyros(3) = decode_32bit(data(251:254),0);

% euler angles
theta_a = decode_32bit(data(287:290),0);
phi_a = decode_32bit(data(291:294),0);

altitude_vision = decode_32bit(data(519:522),0);    %%%% typecast(data(519:522), 'int32');
altitude_vz = decode_32bit(data(523:526),0);
altitude_raw = decode_32bit(data(531:534),0);       %%%% typecast(data(531:534), 'int32');
 
heading_unwrapped = decode_32bit(data(1712:1715),0);
heading_gyro_unwrapped = decode_32bit(data(1716:1719),0);
heading_fusion_unwrapped = decode_32bit(data(1720:1723),0);

magneto_radius = decode_32bit(data(1737:1740),0);
% magneto
mx = decode_16bit(data(1670:1671),1);
my = decode_16bit(data(1672:1673),1);
mz = decode_16bit(data(1674:1675),1);

est_z = decode_32bit(data(1821:1824),0);
est_zdot = decode_32bit(data(1825:1828),0);

%cks
cks = decode_32bit(data(end-3:end),1); 
    
end


function res = decode_32bit(input, mark)
% if mark = 1; then output a int
% else output the float value which is defined by SDK description.
% the input is an array (1*4)
% e.g. : NDS(Battery_OS:Battery_OS+data_length-1)

hex_value = dec2hex(input);
hex_value = [hex_value(4,:),hex_value(3,:),hex_value(2,:),hex_value(1,:)];
if mark ==1
    res = typecast(input,'uint32');%hex2dec(hex_value);
elseif mark ==2
    res = hex2dec(hex_value)-2^31;
else
    res = typecast(input,'single');%typecast(uint32(hex2dec(hex_value)),'single');%
end
res = res(1);
end

function res = decode_16bit(input,mark)
hex_value = dec2hex(input);
hex_value = [hex_value(2,:),hex_value(1,:)];
res = hex2dec(hex_value);
if mark==1
    res=res-2^15;
end
end

function bin = getDroneState(input)
bin = zeros(32,1);
hex = dec2hex(input);
% put the hex_value in the order [31, 30......0]
hex = [hex(4,:),hex(3,:),hex(2,:),hex(1,:)];
for i=1:length(hex)
    if hex(i)=='F'
        bin((i*4)-3:i*4)=[1 1 1 1];
    elseif hex(i)=='E'
        bin((i*4)-3:i*4)=[1 1 1 0];
    elseif hex(i)=='D'
        bin((i*4)-3:i*4)=[1 1 0 1];
    elseif hex(i)=='C'
        bin((i*4)-3:i*4)=[1 1 0 0];
    elseif hex(i)=='B'
        bin((i*4)-3:i*4)=[1 0 1 1];
    elseif hex(i)=='A'
        bin((i*4)-3:i*4)=[1 0 1 0];
    elseif hex(i)=='9'
        bin((i*4)-3:i*4)=[1 0 0 1];
    elseif hex(i)=='8'
        bin((i*4)-3:i*4)=[1 0 0 0];
    elseif hex(i)=='7'
        bin((i*4)-3:i*4)=[0 1 1 1];
    elseif hex(i)=='6'
        bin((i*4)-3:i*4)=[0 1 1 0];
    elseif hex(i)=='5'
        bin((i*4)-3:i*4)=[0 1 0 1];
    elseif hex(i)=='4'
        bin((i*4)-3:i*4)=[0 1 0 0];
    elseif hex(i)=='3'
        bin((i*4)-3:i*4)=[0 0 1 1];
    elseif hex(i)=='2'
        bin((i*4)-3:i*4)=[0 0 1 0];
    elseif hex(i)=='1'
        bin((i*4)-3:i*4)=[0 0 0 1];
    elseif hex(i)=='0'
        bin((i*4)-3:i*4)=[0 0 0 0];
    end
end

end
